simulink model "inversor"  (R2026a)
settings: Solver=VariableStepAuto  MaxStep=1e-3
values from neighbouring files (symbols this model uses):
  Pn_inv = 2000    [inversor_param.m]
  t_delay_com = 0.02    [inversor_param.m]
  tau_pv = 0.5    [inversor_param.m]
libraries: sl_discontinuities x5
settings Model: Creator=arnau.coronado  LastModifiedBy=arnau.coronado

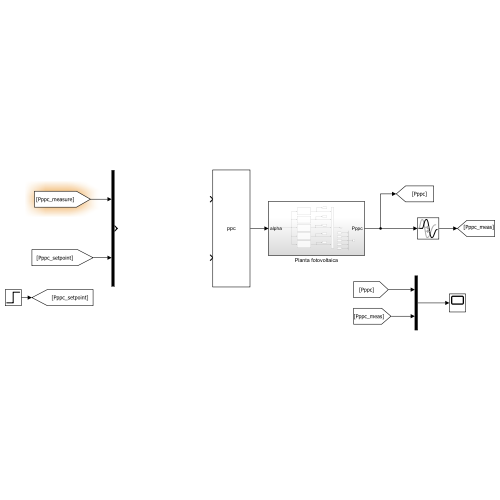
[thumbnail: Simulink's stored preview of the top-level diagram]
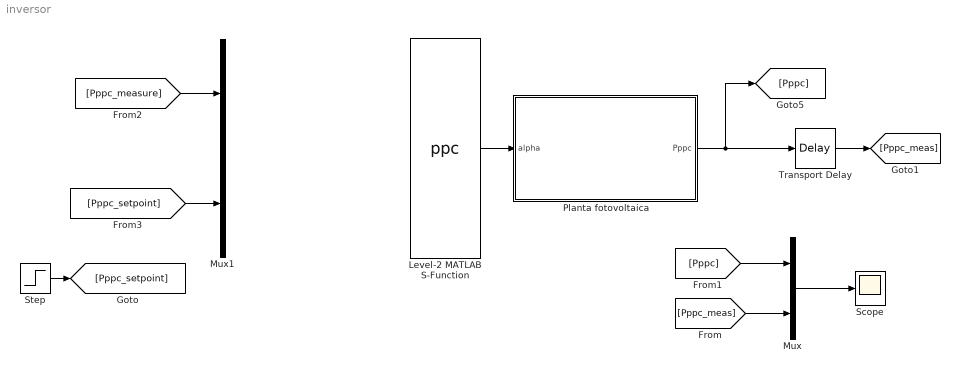
== system inversor ==
  Level-2 MATLAB S-Function : M-S-Function  FunctionName=ppc
  Mux : Mux  Inputs=2
  Mux1 : Mux  Inputs=2
  Planta fotovoltaica : Subsystem
  Scope : Scope
      settings: ActiveDisplayYMinimum=-552.91235244794643  ActiveDisplayYMaximum=12848.577124040576
  Step : Step  SampleTime=0
  Transport Delay : TransportDelay  DelayTime=t_delay_com
  wires:
  Mux/1 -> Scope/1
  [Pppc] -> Mux/1
  [Pppc_meas] -> Mux/2
  Level-2 MATLAB S-Function/1 -> Planta fotovoltaica/1(alpha)
  Planta fotovoltaica/1(Pppc) -> Transport Delay/1, [Pppc]
  Transport Delay/1 -> [Pppc_meas]
  Step/1 -> [Pppc_setpoint]
  [Pppc_setpoint] -> Mux1/2
  [Pppc_measure] -> Mux1/1

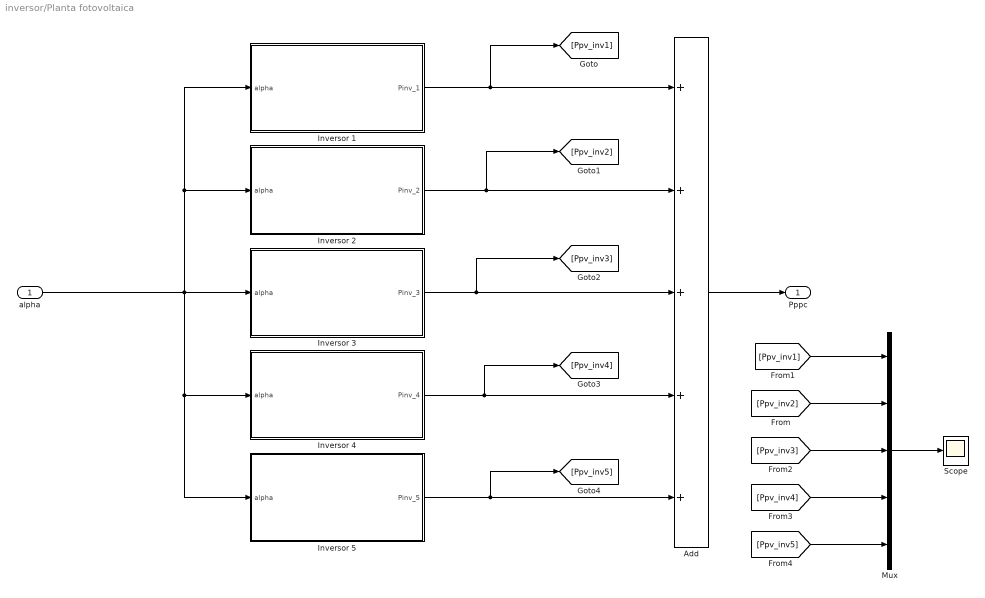
== system inversor/Planta fotovoltaica ==
  alpha : Inport
  Add : Sum  Inputs=+++++
  Inversor 1 : Subsystem
  Inversor 2 : Subsystem
  Inversor 3 : Subsystem
  Inversor 4 : Subsystem
  Inversor 5 : Subsystem
  Mux : Mux  Inputs=5
  Scope : Scope
      settings: ActiveDisplayYMinimum=-264.44761279829225  ActiveDisplayYMaximum=2491.8023717590063
  Pppc : Outport
  wires:
  Inversor 3/1(Pinv_3) -> Add/3, [Ppv_inv3]
  Inversor 2/1(Pinv_2) -> [Ppv_inv2], Add/2
  Inversor 5/1(Pinv_5) -> Add/5, [Ppv_inv5]
  Inversor 4/1(Pinv_4) -> [Ppv_inv4], Add/4
  Inversor 1/1(Pinv_1) -> Add/1, [Ppv_inv1]
  alpha/1 -> Inversor 4/1(alpha), Inversor 5/1(alpha), Inversor 3/1(alpha), Inversor 2/1(alpha), Inversor 1/1(alpha)
  Add/1 -> Pppc/1
  [Ppv_inv5] -> Mux/5
  [Ppv_inv4] -> Mux/4
  Mux/1 -> Scope/1
  [Ppv_inv3] -> Mux/3
  [Ppv_inv2] -> Mux/2
  [Ppv_inv1] -> Mux/1

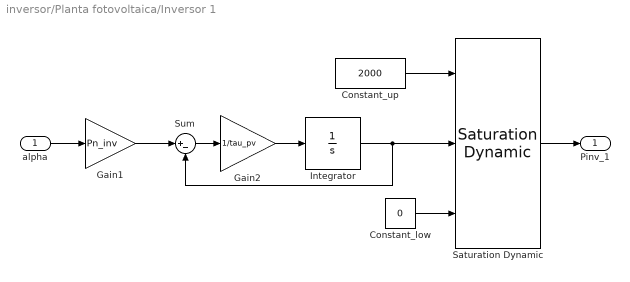
== system inversor/Planta fotovoltaica/Inversor 1 ==
  alpha : Inport
  Constant_low : Constant  Value=0
  Constant_up : Constant  Value=2000
  Gain1 : Gain  Gain=Pn_inv
  Gain2 : Gain  Gain=1/tau_pv
  Integrator : Integrator  InitialCondition=2000
  Saturation Dynamic : sl_discontinuities/Saturation Dynamic  OutMin=[]  OutMax=[]  OutDataTypeStr=Inherit: Same as second input  OutDataType=fixdt(1, 16)  OutScaling=2^-10  DoSatur=off
      settings: LibrarySourceBlock=|
      | simulink/Discontinuities/Saturation
      | Dynamic
  Sum : Sum  Inputs=|+-
  Pinv_1 : Outport
  wires:
  alpha/1 -> Gain1/1
  Integrator/1 -> Sum/2, Saturation Dynamic/2
  Saturation Dynamic/1 -> Pinv_1/1
  Gain1/1 -> Sum/1
  Sum/1 -> Gain2/1
  Constant_low/1 -> Saturation Dynamic/3
  Gain2/1 -> Integrator/1
  Constant_up/1 -> Saturation Dynamic/1

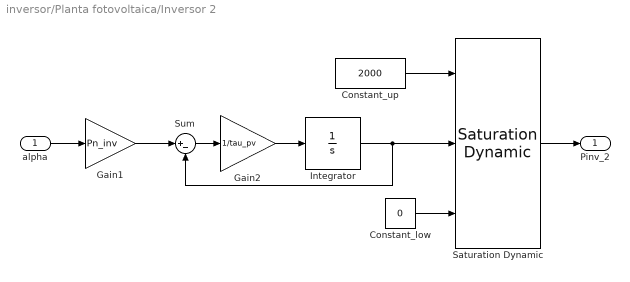
== system inversor/Planta fotovoltaica/Inversor 2 ==
  alpha : Inport
  Constant_low : Constant  Value=0
  Constant_up : Constant  Value=2000
  Gain1 : Gain  Gain=Pn_inv
  Gain2 : Gain  Gain=1/tau_pv
  Integrator : Integrator  InitialCondition=2000
  Saturation Dynamic : sl_discontinuities/Saturation Dynamic  OutMin=[]  OutMax=[]  OutDataTypeStr=Inherit: Same as second input  OutDataType=fixdt(1, 16)  OutScaling=2^-10  DoSatur=off
      settings: LibrarySourceBlock=|
      | simulink/Discontinuities/Saturation
      | Dynamic
  Sum : Sum  Inputs=|+-
  Pinv_2 : Outport
  wires:
  Constant_up/1 -> Saturation Dynamic/1
  Gain2/1 -> Integrator/1
  Constant_low/1 -> Saturation Dynamic/3
  Sum/1 -> Gain2/1
  Gain1/1 -> Sum/1
  Saturation Dynamic/1 -> Pinv_2/1
  Integrator/1 -> Saturation Dynamic/2, Sum/2
  alpha/1 -> Gain1/1

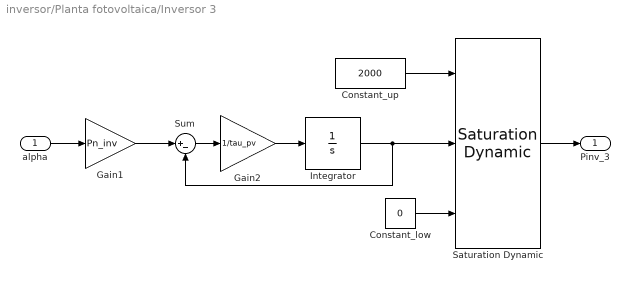
== system inversor/Planta fotovoltaica/Inversor 3 ==
  alpha : Inport
  Constant_low : Constant  Value=0
  Constant_up : Constant  Value=2000
  Gain1 : Gain  Gain=Pn_inv
  Gain2 : Gain  Gain=1/tau_pv
  Integrator : Integrator  InitialCondition=2000
  Saturation Dynamic : sl_discontinuities/Saturation Dynamic  OutMin=[]  OutMax=[]  OutDataTypeStr=Inherit: Same as second input  OutDataType=fixdt(1, 16)  OutScaling=2^-10  DoSatur=off
      settings: LibrarySourceBlock=|
      | simulink/Discontinuities/Saturation
      | Dynamic
  Sum : Sum  Inputs=|+-
  Pinv_3 : Outport
  wires:
  alpha/1 -> Gain1/1
  Integrator/1 -> Sum/2, Saturation Dynamic/2
  Saturation Dynamic/1 -> Pinv_3/1
  Gain1/1 -> Sum/1
  Sum/1 -> Gain2/1
  Constant_low/1 -> Saturation Dynamic/3
  Gain2/1 -> Integrator/1
  Constant_up/1 -> Saturation Dynamic/1

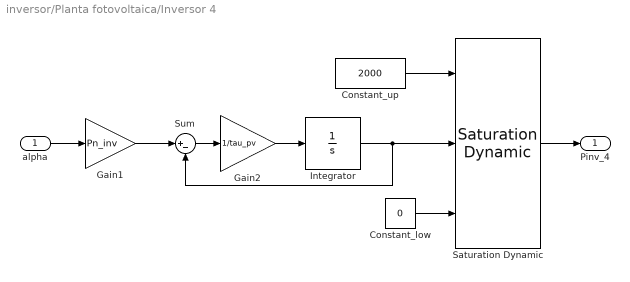
== system inversor/Planta fotovoltaica/Inversor 4 ==
  alpha : Inport
  Constant_low : Constant  Value=0
  Constant_up : Constant  Value=2000
  Gain1 : Gain  Gain=Pn_inv
  Gain2 : Gain  Gain=1/tau_pv
  Integrator : Integrator  InitialCondition=2000
  Saturation Dynamic : sl_discontinuities/Saturation Dynamic  OutMin=[]  OutMax=[]  OutDataTypeStr=Inherit: Same as second input  OutDataType=fixdt(1, 16)  OutScaling=2^-10  DoSatur=off
      settings: LibrarySourceBlock=|
      | simulink/Discontinuities/Saturation
      | Dynamic
  Sum : Sum  Inputs=|+-
  Pinv_4 : Outport
  wires:
  Constant_up/1 -> Saturation Dynamic/1
  Gain2/1 -> Integrator/1
  Constant_low/1 -> Saturation Dynamic/3
  Sum/1 -> Gain2/1
  Gain1/1 -> Sum/1
  Saturation Dynamic/1 -> Pinv_4/1
  Integrator/1 -> Saturation Dynamic/2, Sum/2
  alpha/1 -> Gain1/1

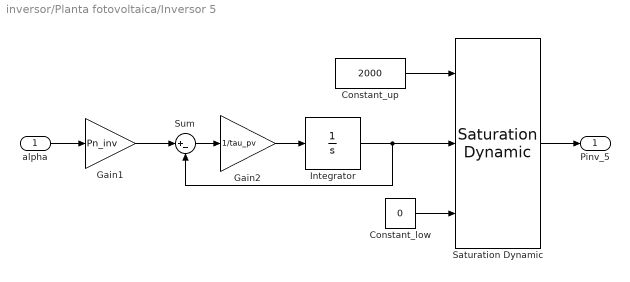
== system inversor/Planta fotovoltaica/Inversor 5 ==
  alpha : Inport
  Constant_low : Constant  Value=0
  Constant_up : Constant  Value=2000
  Gain1 : Gain  Gain=Pn_inv
  Gain2 : Gain  Gain=1/tau_pv
  Integrator : Integrator  InitialCondition=2000
  Saturation Dynamic : sl_discontinuities/Saturation Dynamic  OutMin=[]  OutMax=[]  OutDataTypeStr=Inherit: Same as second input  OutDataType=fixdt(1, 16)  OutScaling=2^-10  DoSatur=off
      settings: LibrarySourceBlock=|
      | simulink/Discontinuities/Saturation
      | Dynamic
  Sum : Sum  Inputs=|+-
  Pinv_5 : Outport
  wires:
  alpha/1 -> Gain1/1
  Integrator/1 -> Sum/2, Saturation Dynamic/2
  Saturation Dynamic/1 -> Pinv_5/1
  Gain1/1 -> Sum/1
  Sum/1 -> Gain2/1
  Constant_low/1 -> Saturation Dynamic/3
  Gain2/1 -> Integrator/1
  Constant_up/1 -> Saturation Dynamic/1
